simulink model "p1_4_quick_release"  (R2025b)
settings: Solver=ode45  StartTime=0.0  StopTime=2  MaxStep=2e-4  RelTol=1e-7
values from neighbouring files (symbols this model uses):
  mp = block.DialogPrm(2).Data    [m01_anim.m]    (also in m01_params.m = [])
  tq = 1    [p1_4_quick_release.m]    (also in p1_5_mass_sweep.m; p1_6_series_elasticity.m)
undefined symbols (not defined in the file or in its folder): m_load
settings Model: Creator=maria  LastModifiedBy=maria

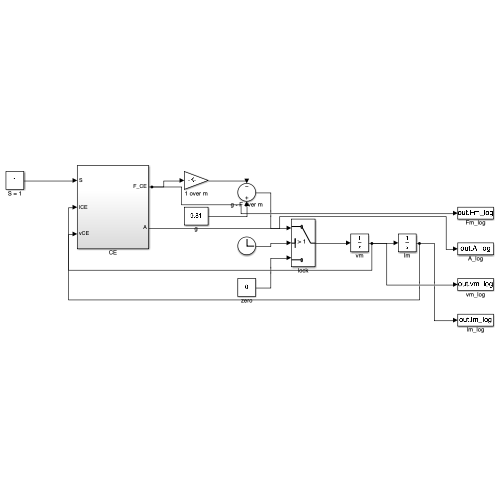
[thumbnail: Simulink's stored preview of the top-level diagram]
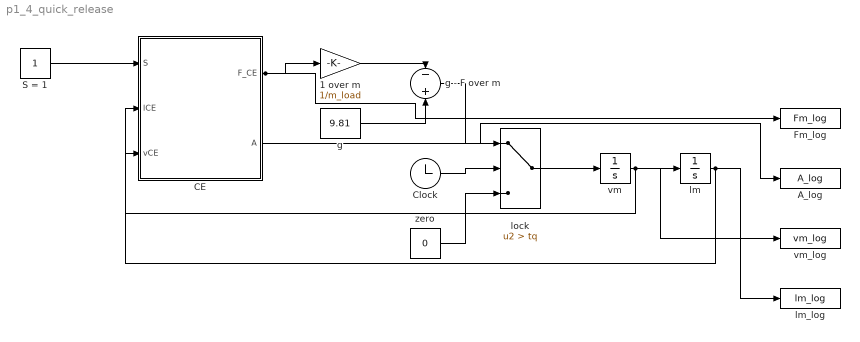
== system p1_4_quick_release ==
  1 over m : Gain  Gain=1/m_load
  A_log : ToWorkspace  VariableName=A_log  SaveFormat=Timeseries  SampleTime=-1
  CE : Subsystem
  Clock : Clock
  Fm_log : ToWorkspace  VariableName=Fm_log  SaveFormat=Timeseries  SampleTime=-1
  S = 1 : Constant
  g : Constant  Value=9.81
  g - F over m : Sum  Inputs=-+
  lm : Integrator  InitialCondition=mp.lopt
  lm_log : ToWorkspace  VariableName=lm_log  SaveFormat=Timeseries  SampleTime=-1
  lock : Switch  Criteria=u2 > Threshold  Threshold=tq  SaturateOnIntegerOverflow=off  InputSameDT=off
  vm : Integrator
  vm_log : ToWorkspace  VariableName=vm_log  SaveFormat=Timeseries  SampleTime=-1
  zero : Constant  Value=0
  wires:
  S = 1/1 -> CE/1(S)
  CE/1(F_CE) -> 1 over m/1, Fm_log/1
  1 over m/1 -> g - F over m/1
  g/1 -> g - F over m/2
  g - F over m/1 -> lock/1
  Clock/1 -> lock/2
  zero/1 -> lock/3
  lock/1 -> vm/1
  vm/1 -> lm/1, CE/3(vCE), vm_log/1
  lm/1 -> CE/2(lCE), lm_log/1
  CE/2(A) -> A_log/1

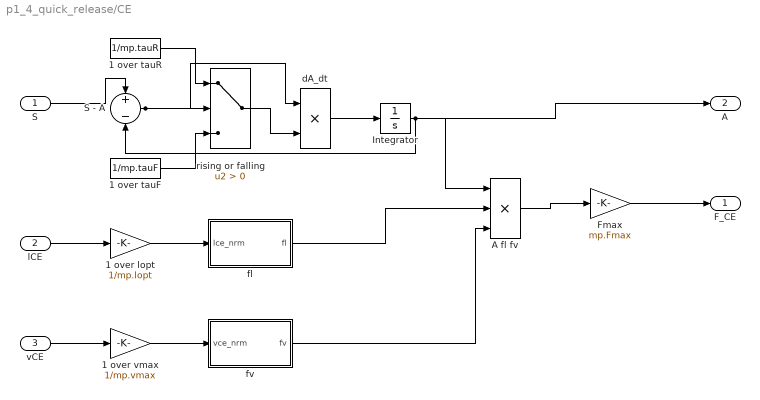
== system p1_4_quick_release/CE ==
  S : Inport
  lCE : Inport  Port=2
  vCE : Inport  Port=3
  1 over lopt : Gain  Gain=1/mp.lopt
  1 over tauF : Constant  Value=1/mp.tauF
  1 over tauR : Constant  Value=1/mp.tauR
  1 over vmax : Gain  Gain=1/mp.vmax
  A fl fv : Product  Inputs=3
  Fmax : Gain  Gain=mp.Fmax
  Integrator : Integrator  InitialCondition=mp.A0
  S - A : Sum  Inputs=+-
  dA_dt : Product
  fl : MATLAB Function  TreatAsAtomicUnit=on
  fv : MATLAB Function  TreatAsAtomicUnit=on
  rising or falling : Switch  Criteria=u2 > Threshold  SaturateOnIntegerOverflow=off  InputSameDT=off
  F_CE : Outport
  A : Outport  Port=2
  wires:
  S/1 -> S - A/1
  Integrator/1 -> S - A/2, A/1, A fl fv/1
  S - A/1 -> rising or falling/2, dA_dt/1
  1 over tauR/1 -> rising or falling/1
  1 over tauF/1 -> rising or falling/3
  rising or falling/1 -> dA_dt/2
  dA_dt/1 -> Integrator/1
  lCE/1 -> 1 over lopt/1
  vCE/1 -> 1 over vmax/1
  1 over lopt/1 -> fl/1(lce_nrm)
  1 over vmax/1 -> fv/1(vce_nrm)
  fl/1(fl) -> A fl fv/2
  fv/1(fv) -> A fl fv/3
  A fl fv/1 -> Fmax/1
  Fmax/1 -> F_CE/1

== matlab function p1_4_quick_release/CE/fl ==
  data: lce_nrm input; fl output; mp parameter
function fl = fcn(lce_nrm, mp)
fl = CE_force_length_relation(lce_nrm, mp);

== matlab function p1_4_quick_release/CE/fv ==
  data: vce_nrm input; fv output; mp parameter
function fv = fcn(vce_nrm, mp)
fv = CE_force_velocity_relation(vce_nrm, mp);
